simulink model "batterychargerfyp"  (R2022b)
settings: Solver=VariableStepAuto  StartTime=0.0  StopTime=1  RelTol=1e-3
undefined symbols (not defined in the file or in its folder): Ion, Lithium
libraries: spsThyristorLib x6, spsSeriesRLCBranchLib x3, slpidlib x2, spsVoltageMeasurementLib x2, spsBatteryLib x1, spsCurrentMeasurementLib x1, spsDiodeLib x1, spsGroundLib x1, spsMosfetLib x1, spsParallelRLCBranchLib x1, spsSawtoothGeneratorLib x1, spsThreePhaseVIMeasurementLib x1
settings Model: Creator=Aoun Raza  LastModifiedBy=Aoun Raza

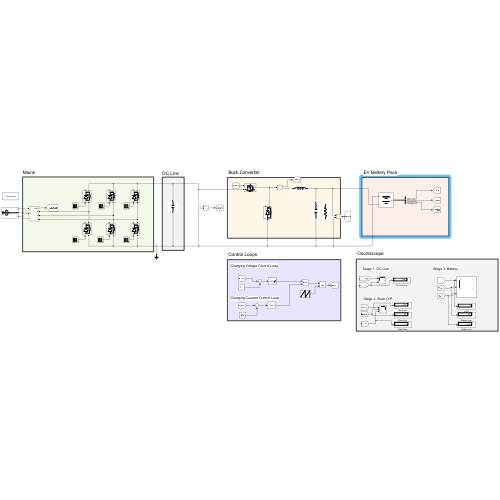
[thumbnail: Simulink's stored preview of the top-level diagram]
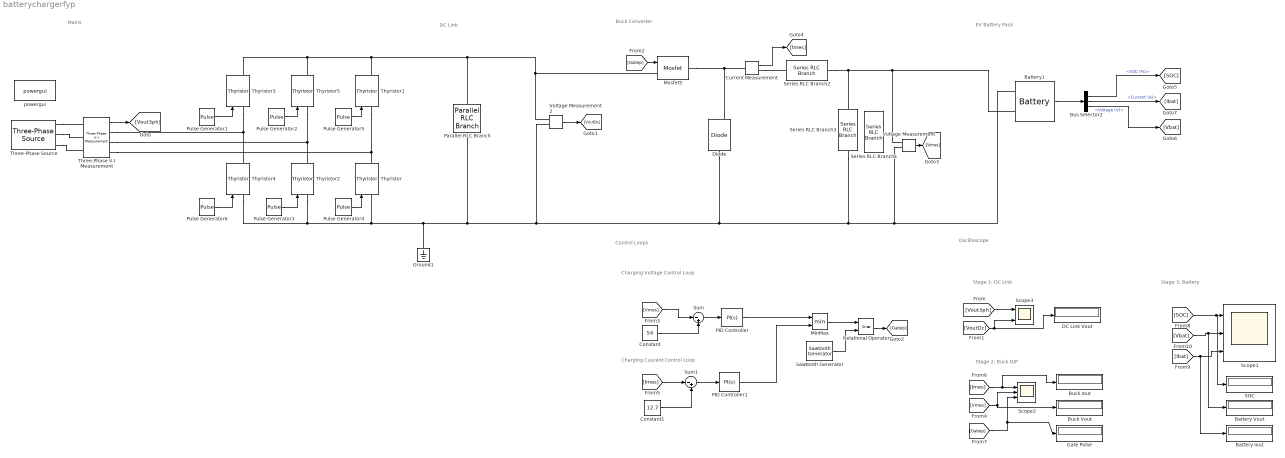
== system batterychargerfyp ==
  note: Control Loops
  note: Stage 1: DC Link
  note: Oscilloscope
  note: Charging Voltage Control Loop
  note: Mains
  note: DC Link
  note: EV Battery Pack
  note: Buck Converter
  note: Stage 2: Buck O/P
  note: Charging Cuurent Control Loop
  note: Stage 3: Battery
  Battery Iout : Display
  Battery Vout : Display
  Battery1 : spsBatteryLib/Battery  BatType=Lithium-Ion  ShowTempParam=off  ThermalPreset=no  ShowAgeParam=off  NomV=48  NomQ=18  SOC=50  Batt_Tr=10  PresetModel=on  MaxQ=18  MinV=36  FullV=55.8714  Dis_rate=7.8261  R=0.026667  Normal_OP=16.2783  expZone="[51.8585     0.884348]"  current=[6.5 13 32.5]  Units=Time  Tci=20  NomT=20  T2=-30  MaxQ2=4.8  FullV2=7.1  Normal_OP2=5.655  expZone2="[6.58           1]"  Rca=0.6  ti=2000  Dp=0  Neq0=0  Tsim=1e6  Ta1=25  Qeol=5.4*0.9  Reol=0.013333*1.2  Char_age=[2.3478, 3]  Dis_age=[2.3478, 10]  N1=1500  N2=10500  N3=1000  N4=1400  Ta2=45  N5=950
  Buck Iout : Display
  Buck Vout : Display
  Bus Selector2 : BusSelector  OutputSignals=SOC (%),Current (A),Voltage (V)
  Constant : Constant  Value=54
  Constant1 : Constant  Value=12.7
  Current Measurement : spsCurrentMeasurementLib/Current Measurement  PhasorSimulation=off  OutputType=Complex  PSBequivalent=0
  DC Link Vout : Display
  Diode : spsDiodeLib/Diode  Ron=0.001  Lon=0  Vf=0.8  IC=0  UseSnubber=0  Rs=500  Cs=250e-9  Measurements=on
  Gate Pulse : Display
  Ground1 : spsGroundLib/Ground  LConnTagsString=a
  MinMax : MinMax  Inputs=2
  Mosfet5 : spsMosfetLib/Mosfet  Ron=0.1  Lon=0  Rd=0.01  Vfd=0  IC=0  Rs=1e5  Cs=inf  Measurements=off
  PID Controller : slpidlib/PID Controller  Controller=PI  Form=Parallel  TimeDomain=Continuous-time  UseExternalTs=off  SampleTime=-1  IntegratorMethod=Forward Euler  FilterMethod=Forward Euler  ControllerParametersSource=internal  P=0.05  I=5  UseKiTs=off  D=0  N=100  UseFilter=on  TunerSelectOption=Transfer Function Based (PID Tuner App)  InitialConditionSource=internal  InitialConditionForIntegrator=0  InitialConditionForFilter=0  DifferentiatorICPrevScaledInput=0  ExternalReset=none  TrackingMode=off  Kt=1  LimitOutput=on  SatLimitsSource=internal  UpperSaturationLimit=0.9  LowerSaturationLimit=0  LinearizeAsGain=on  AntiWindupMode=none  Kb=1  LimitIntegrator=off  UpperIntegratorSaturationLimit=inf  LowerIntegratorSaturationLimit=-inf  POutMin=[]  POutMax=[]  IOutMin=[]  IOutMax=[]  DOutMin=[]  DOutMax=[]  NOutMin=[]  NOutMax=[]  SumOutMin=[]  SumOutMax=[]  SaturationOutMin=[]  SaturationOutMax=[]  PParamMin=[]  PParamMax=[]  IParamMin=[]  IParamMax=[]  DParamMin=[]  DParamMax=[]  NParamMin=[]  NParamMax=[]  KbParamMin=[]  KbParamMax=[]  KtParamMin=[]  KtParamMax=[]  KbOutMin=[]  KbOutMax=[]  KtOutMin=[]  KtOutMax=[]  IntegratorOutMin=[]  IntegratorOutMax=[]  FilterOutMin=[]  FilterOutMax=[]  SumI1OutMin=[]  SumI1OutMax=[]  SumI2OutMin=[]  SumI2OutMax=[]  SumI3OutMin=[]  SumI3OutMax=[]  SumI4OutMin=[]  SumI4OutMax=[]  SumDOutMin=[]  SumDOutMax=[]  DifferentiatorOutMin=[]  DifferentiatorOutMax=[]  FilterDiffOutCoefMin=[]  FilterDiffOutCoefMax=[]  ReciprocalOutMin=[]  ReciprocalOutMax=[]  SumDenOutMin=[]  SumDenOutMax=[]  SumNumOutMin=[]  SumNumOutMax=[]  DivideOutMin=[]  DivideOutMax=[]  UdiffTsProdOutMin=[]  UdiffTsProdOutMax=[]  NTsProdOutMin=[]  NTsProdOutMax=[]  UintegralTsProdOutMin=[]  UintegralTsProdOutMax=[]  UngainTsProdOutMin=[]  UngainTsProdOutMax=[]  ClampingZeroOutDataTypeStr=Inherit: Inherit via back propagation  ClampingZeroOutMin=[]  ClampingZeroOutMax=[]  FilterDenConstantOutDataTypeStr=Inherit: Inherit via back propagation  FilterDenConstantOutMin=[]  FilterDenConstantOutMax=[]  PCopyOutDataTypeStr=Inherit: Inherit via back propagation  PCopyOutMin=[]  PCopyOutMax=[]  NCopyOutDataTypeStr=Inherit: Inherit via back propagation  NCopyOutMin=[]  NCopyOutMax=[]  IntegratorContinuousStateAttributes=''  IntegratorStateMustResolveToSignalObject=off  IntegratorRTWStateStorageClass=Auto  FilterContinuousStateAttributes=''  FilterStateMustResolveToSignalObject=off  FilterRTWStateStorageClass=Auto  ParallelPVariant=InternalParameters  IdealPVariant=Disabled  IVariant=InternalParameters  DVariant=Disabled  IntegratorVariant=Continuous  SatVariant=Enabled  AWVariant=Passthrough  PCopyVariant=Disabled  TRVariant=Disabled  FdbkBlocksVariant=Forward  IdealPFdbkVariant=Disabled  SatFdbkVariant=Disabled  DerivativeFilterVariant=Disabled  NVariant=Disabled  NCopyVariant=Disabled_SignalSpec  FilterICVariant=Disabled  IntegratorICVariant=InternalICs  ExternalResetVariant=Disabled  TRSumVariant=Passthrough  SumFdbkVariant=Disabled  SumVariant=Sum_PI  TsampFilterVariant=InternalTs  TsampNgainVariant=Passthrough  TsampIntegralVariant=Passthrough  ExternalSaturationOutDataTypeStr=Inherit: Same as second input
  PID Controller1 : slpidlib/PID Controller  Controller=PI  Form=Parallel  TimeDomain=Continuous-time  UseExternalTs=off  SampleTime=-1  IntegratorMethod=Forward Euler  FilterMethod=Forward Euler  ControllerParametersSource=internal  P=0.02  I=5  UseKiTs=off  D=0  N=100  UseFilter=on  TunerSelectOption=Transfer Function Based (PID Tuner App)  InitialConditionSource=internal  InitialConditionForIntegrator=0  InitialConditionForFilter=0  DifferentiatorICPrevScaledInput=0  ExternalReset=none  TrackingMode=off  Kt=1  LimitOutput=off  SatLimitsSource=internal  UpperSaturationLimit=inf  LowerSaturationLimit=-inf  LinearizeAsGain=on  AntiWindupMode=none  Kb=1  LimitIntegrator=off  UpperIntegratorSaturationLimit=inf  LowerIntegratorSaturationLimit=-inf  POutMin=[]  POutMax=[]  IOutMin=[]  IOutMax=[]  DOutMin=[]  DOutMax=[]  NOutMin=[]  NOutMax=[]  SumOutMin=[]  SumOutMax=[]  SaturationOutMin=[]  SaturationOutMax=[]  PParamMin=[]  PParamMax=[]  IParamMin=[]  IParamMax=[]  DParamMin=[]  DParamMax=[]  NParamMin=[]  NParamMax=[]  KbParamMin=[]  KbParamMax=[]  KtParamMin=[]  KtParamMax=[]  KbOutMin=[]  KbOutMax=[]  KtOutMin=[]  KtOutMax=[]  IntegratorOutMin=[]  IntegratorOutMax=[]  FilterOutMin=[]  FilterOutMax=[]  SumI1OutMin=[]  SumI1OutMax=[]  SumI2OutMin=[]  SumI2OutMax=[]  SumI3OutMin=[]  SumI3OutMax=[]  SumI4OutMin=[]  SumI4OutMax=[]  SumDOutMin=[]  SumDOutMax=[]  DifferentiatorOutMin=[]  DifferentiatorOutMax=[]  FilterDiffOutCoefMin=[]  FilterDiffOutCoefMax=[]  ReciprocalOutMin=[]  ReciprocalOutMax=[]  SumDenOutMin=[]  SumDenOutMax=[]  SumNumOutMin=[]  SumNumOutMax=[]  DivideOutMin=[]  DivideOutMax=[]  UdiffTsProdOutMin=[]  UdiffTsProdOutMax=[]  NTsProdOutMin=[]  NTsProdOutMax=[]  UintegralTsProdOutMin=[]  UintegralTsProdOutMax=[]  UngainTsProdOutMin=[]  UngainTsProdOutMax=[]  ClampingZeroOutDataTypeStr=Inherit: Inherit via back propagation  ClampingZeroOutMin=[]  ClampingZeroOutMax=[]  FilterDenConstantOutDataTypeStr=Inherit: Inherit via back propagation  FilterDenConstantOutMin=[]  FilterDenConstantOutMax=[]  PCopyOutDataTypeStr=Inherit: Inherit via back propagation  PCopyOutMin=[]  PCopyOutMax=[]  NCopyOutDataTypeStr=Inherit: Inherit via back propagation  NCopyOutMin=[]  NCopyOutMax=[]  IntegratorContinuousStateAttributes=''  IntegratorStateMustResolveToSignalObject=off  IntegratorRTWStateStorageClass=Auto  FilterContinuousStateAttributes=''  FilterStateMustResolveToSignalObject=off  FilterRTWStateStorageClass=Auto  ParallelPVariant=InternalParameters  IdealPVariant=Disabled  IVariant=InternalParameters  DVariant=Disabled  IntegratorVariant=Continuous  SatVariant=Disabled  AWVariant=Passthrough  PCopyVariant=Disabled  TRVariant=Disabled  FdbkBlocksVariant=Forward  IdealPFdbkVariant=Disabled  SatFdbkVariant=Disabled  DerivativeFilterVariant=Disabled  NVariant=Disabled  NCopyVariant=Disabled_SignalSpec  FilterICVariant=Disabled  IntegratorICVariant=InternalICs  ExternalResetVariant=Disabled  TRSumVariant=Passthrough  SumFdbkVariant=Disabled  SumVariant=Sum_PI  TsampFilterVariant=InternalTs  TsampNgainVariant=Passthrough  TsampIntegralVariant=Passthrough  ExternalSaturationOutDataTypeStr=Inherit: Same as second input
  Parallel RLC Branch : spsParallelRLCBranchLib/Parallel RLC Branch  LConnTagsString=a  RConnTagsString=__new0  BranchType=C  Resistance=1  Inductance=1e-3  SetiL0=off  InitialCurrent=0  Capacitance=1000e-6  Setx0=off  InitialVoltage=0  Measurements=None
  Pulse Generator1 : DiscretePulseGenerator  PulseType=Time based  Period=0.02  PulseWidth=10  PhaseDelay=(0)*0.02/360
  Pulse Generator2 : DiscretePulseGenerator  PulseType=Time based  Period=0.02  PulseWidth=10  PhaseDelay=(120)*0.02/360
  Pulse Generator3 : DiscretePulseGenerator  PulseType=Time based  Period=0.02  PulseWidth=10  PhaseDelay=(300)*0.02/360
  Pulse Generator4 : DiscretePulseGenerator  PulseType=Time based  Period=0.02  PulseWidth=10  PhaseDelay=(60)*0.02/360
  Pulse Generator5 : DiscretePulseGenerator  PulseType=Time based  Period=0.02  PulseWidth=10  PhaseDelay=(240)*0.02/360
  Pulse Generator6 : DiscretePulseGenerator  PulseType=Time based  Period=0.02  PulseWidth=10  PhaseDelay=(180)*0.02/360
  Relational Operator : RelationalOperator  OutDataTypeStr=boolean  RndMeth=Simplest  InputSameDT=off
  SOC : Display
  Sawtooth Generator : spsSawtoothGeneratorLib/Sawtooth Generator  Freq=20000  Phase=0  Ts=0
  Scope1 : Scope  NumInputPorts=3
  Scope2 : Scope  NumInputPorts=3
  Scope3 : Scope  NumInputPorts=2
  Series RLC Branch1 : spsSeriesRLCBranchLib/Series RLC Branch  LConnTagsString=__new0  RConnTagsString=__new0  BranchType=R  Resistance=2000  Inductance=1e-3  SetiL0=off  InitialCurrent=0  Capacitance=1000e-6  Setx0=off  InitialVoltage=0  Measurements=None
  Series RLC Branch2 : spsSeriesRLCBranchLib/Series RLC Branch  LConnTagsString=__new0  RConnTagsString=__new0  BranchType=L  Resistance=1  Inductance=1.5e-3  SetiL0=off  InitialCurrent=0  Capacitance=1e-6  Setx0=off  InitialVoltage=0  Measurements=None
  Series RLC Branch3 : spsSeriesRLCBranchLib/Series RLC Branch  LConnTagsString=__new0  RConnTagsString=__new0  BranchType=C  Resistance=2000  Inductance=1e-3  SetiL0=off  InitialCurrent=0  Capacitance=1000e-6  Setx0=off  InitialVoltage=0  Measurements=None
  Sum : Sum  Inputs=|-+
  Sum1 : Sum  Inputs=|-+
  Three-Phase V-I Measurement : spsThreePhaseVIMeasurementLib/Three-Phase V-I Measurement  VoltageMeasurement=phase-to-phase  SetLabelV=off  LabelV=Vabc  Vpu=off  VpuLL=off  CurrentMeasurement=no  SetLabelI=off  LabelI=Iabc  Ipu=off  Pbase=100e6  Vbase=500e3  OutputType=Complex  PhasorSimulation=off  PSBequivalent=0
  Three-Phase Source : spsThreePhaseSourceLib/Three-Phase Source  InternalConnection=Yg  VoltagePhases=off  Voltage=220  PhaseAngle=0  Voltage_phases=[25e3 25e3 25e3]/sqrt(3)  PhaseAngles_phases=[0 -120 +120]  Frequency=50  NonIdealSource=off  SpecifyImpedance=off  Resistance=0.8929  Inductance=16.58e-3  ShortCircuitLevel=100e6  BaseVoltage=25e3  XRratio=7  BusType=swing  Pref=10e3  Qref=0  Prefabc=[10e3, 10e3, 10e3]  Qrefabc=[0, 0, 0]  Qmin=-inf  Qmax=inf
  Thyristor{,1..5} (6 alike) : spsThyristorLib/Thyristor  Ron=0.001  Lon=0  Vf=0.8  IC=0  Rs=500  Cs=250e-9  Measurements=on
  Voltage Measurement : spsVoltageMeasurementLib/Voltage Measurement  PhasorSimulation=off  OutputType=Complex  PSBequivalent=0
  Voltage Measurement2 : spsVoltageMeasurementLib/Voltage Measurement  PhasorSimulation=off  OutputType=Complex  PSBequivalent=0
  powergui : spspowerguiLib/powergui  Priority=1  SimulationMode=Continuous  SampleTime=50e-6  frequency=60  Iterations=50  frequencyindice=0  Pbase=100e6  ErrMax=1e-4  UnitsV=kV  UnitsW=MW  buscounter=0  FunctionMessages=off  echomessages=off  EnableUseOfTLC=off  CurrentSourceSwitches=off  DisableSnubberDevices=off  DisableRonSwitches=off  DisableVfSwitches=off  DisplayEquations=off  AutomaticDiscreteSolvers=off  SolverType=Tustin/Backward Euler (TBE)  Interpol=off  ExternalGateDelay=off  methode=off  Ts=100  x0status=blocks  SPID=on  SwTol=0  HookPort=off  NonlinearTolerance=1e-4  nMaxIteration=100  ContinueOnMaxIteration=off  RestoreLinks=warning  ResistiveCurrentMeasurement=off  Frange=[0:2:500]  Ylog=off  Xlog=on  ShowGrid=off  save=off  variable=ZData  structure=0  ZoomFFT=off  StartTime=0.0  cycles=1  DisplayStyle=1  fundamental=60  FreqAxis=off  MaxFrequency=1000  frequencyindicesteady=1  RmsSteady=1  display=off
  wires:
  Battery1/1 -> Bus Selector2/1
  Bus Selector2/1 -> [SOC]  "<SOC (%)>"
  Bus Selector2/3 -> [Vbat]  "<Voltage (V)>"
  Bus Selector2/2 -> [Ibat]  "<Current (A)>"
  Pulse Generator1/1 -> Thyristor3/1
  Pulse Generator4/1 -> Thyristor/1
  Pulse Generator2/1 -> Thyristor5/1
  Pulse Generator6/1 -> Thyristor4/1
  Pulse Generator5/1 -> Thyristor1/1
  Pulse Generator3/1 -> Thyristor2/1
  Three-Phase V-I Measurement/1 -> [Vout3ph]
  Current Measurement/1 -> [Imes]
  Voltage Measurement/1 -> [Vmes]
  Constant/1 -> Sum/2
  Sum/1 -> PID Controller/1
  Constant1/1 -> Sum1/2
  Sum1/1 -> PID Controller1/1
  PID Controller1/1 -> MinMax/2
  Sawtooth Generator/1 -> Relational Operator/2
  Relational Operator/1 -> [Gateip]
  [Vout3ph] -> Scope3/1
  Voltage Measurement2/1 -> [VoutDc]
  [VoutDc] -> DC Link Vout/1, Scope3/2
  [Gateip] -> Mosfet5/1
  [Vmes] -> Sum/1
  [Vmes] -> Buck Vout/1, Scope2/2
  [Imes] -> Buck Iout/1, Scope2/1
  PID Controller/1 -> MinMax/1
  MinMax/1 -> Relational Operator/1
  [Imes] -> Sum1/1
  [Gateip] -> Scope2/3, Gate Pulse/1
  [SOC] -> SOC/1, Scope1/1
  [Vbat] -> Battery Vout/1, Scope1/2
  [Ibat] -> Battery Iout/1, Scope1/3
  connections:
  Three-Phase Source/RConn1 -- Three-Phase V-I Measurement/LConn1
  Three-Phase Source/RConn2 -- Three-Phase V-I Measurement/LConn2
  Three-Phase Source/RConn3 -- Three-Phase V-I Measurement/LConn3
  Thyristor3/RConn1 -- Thyristor5/RConn1 -- Voltage Measurement2/LConn1 -- Mosfet5/LConn1 -- Parallel RLC Branch/LConn1 -- Thyristor1/RConn1
  Thyristor3/LConn1 -- Thyristor4/RConn1 -- Three-Phase V-I Measurement/RConn1
  Thyristor5/LConn1 -- Thyristor2/RConn1 -- Three-Phase V-I Measurement/RConn2
  Thyristor1/LConn1 -- Three-Phase V-I Measurement/RConn3 -- Thyristor/RConn1
  Diode/RConn1 -- Mosfet5/RConn1 -- Current Measurement/LConn1
  Current Measurement/RConn1 -- Series RLC Branch2/LConn1
  Diode/LConn1 -- Voltage Measurement/LConn2 -- Battery1/LConn2 -- Series RLC Branch3/RConn1 -- Voltage Measurement2/LConn2 -- Ground1/LConn1 -- Thyristor/LConn1 -- Thyristor2/LConn1 -- Thyristor4/LConn1 -- Parallel RLC Branch/RConn1
  Series RLC Branch2/RConn1 -- Voltage Measurement/LConn1 -- Battery1/LConn1 -- Series RLC Branch3/LConn1
